simulink model "ADC_forumkerhuel_OC_HW_Fs30k_PIC32"  (Simulink 7.2)
settings: Solver=FixedStepDiscrete  StartTime=0.0  StopTime=inf  FixedStep=1/30000  RelTol=1e-3
undefined symbols (not defined in the file or in its folder): ANmax, OCmax
libraries: dsPICdrivers x4
settings Model: Creator=Lubin  LastModifiedBy=Casparus  BufferReuse=off
settings OptimizationCC: BlockReduction=off  OptimizeBlockIOStorage=off  BufferReuse=off  ExpressionFolding=off  LocalBlockOutputs=off  InitFltsAndDblsToZero=on  OptimizeModelRefInitCode=on  LifeSpan=1
settings DebuggingCC: SaveWithParameterizedLinksMsg=none  SignalResolutionControl=TryResolveAllWithWarning  InheritedTsInSrcMsg=none  IntegerOverflowMsg=none  ParameterOverflowMsg=none
settings HardwareCC: TargetHWDeviceType=32-bit Generic
settings RTWCC: SystemTargetFile=pic32.tlc  TemplateMakefile=pic32_gcc.tmf  PostCodeGenCommand=dsPIC_Compile()  Description=Embedded Target for Microchip dsPIC (real-time)  ProcessScript=pic32_make_rtw_hook
settings CodeAppCC: IgnoreCustomStorageClasses=off
settings STFCustomTargetCC: ModelReferenceCompliant=off  IncludeMdlTerminateFcn=off  CombineOutputUpdateFcns=on  SuppressErrorStatus=on  ERTCustomFileBanners=on  SupportContinuousTime=off  SupportNonInlinedSFcns=off  SystemTargetFile=pic32.tlc
settings ERTTargetCC: MultiwordLength=2048  ModelReferenceCompliant=off  CompOptLevelCompliant=off  IncludeMdlTerminateFcn=off  SuppressErrorStatus=on  ERTFirstTimeCompliant=off  ModelStepFunctionPrototypeControlCompliant=off  CPPClassGenCompliant=off  InlinedParameterPlacement=NonHierarchical  ERTSrcFileBannerTemplate=dsPIC_code_template.cgt  ERTHdrFileBannerTemplate=dsPIC_code_template.cgt  ERTDataSrcFileTemplate=dsPIC_code_template.cgt  ERTDataHdrFileTemplate=dsPIC_code_template.cgt  ERTCustomFileTemplate=dsPIC_main.tlc
settings CustomProperty: DataType=string  Value=C:\PROGRA~1\MATLAB\R2008b\bin\win32\gmake

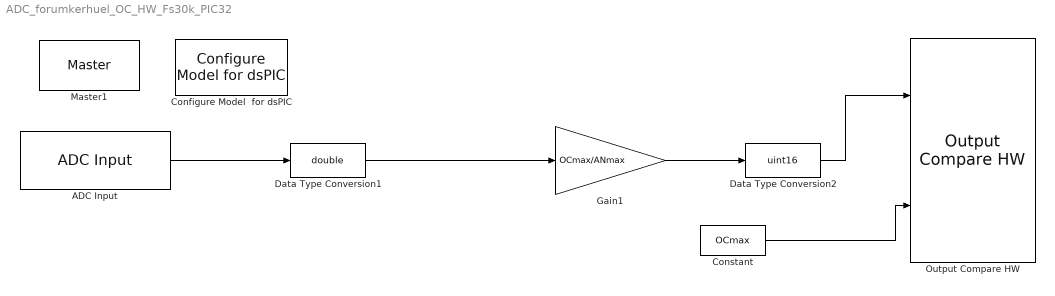
== system ADC_forumkerhuel_OC_HW_Fs30k_PIC32 ==
  ADC Input : dsPICdrivers/Peripheral I//O/ADC Input  Tag=dsPIC_ADC  Priority=5  ADC_TYPE=10 bits  ADC_MODE=Continuous sampling & get last channel value  NbrSampleStep=1  VoltRefpopup="AVdd  -  AVss"  OutFormatBitspopup=0000 00dd dddd dddd : Integer  InterruptPriority=7  ANCHANNELS=[0]  MaxName=ANmax = 1023  Rin=1e2  ADCS=12  SAMC=1  Temperature=25  DMAChannel=0  SampleTime=1/30000  Status="OK  |  Tsmp=1.625e-007 |  T/Channel=2.113e-006 |  Tall=2.113e-006"  SSRC=Timer3 (OC_HW PWM)
  Configure Model  for dsPIC : dsPICdrivers/Simulink Configuration/Configure Model  for dsPIC
  Constant : Constant  Value=OCmax  OutDataTypeMode=uint16  OutDataType=sfix(16)  OutScaling=2^0  OutDataTypeStr=uint16
  Data Type Conversion1 : DataTypeConversion  OutDataTypeMode=double  OutDataType=sfix(16)  OutScaling=2^0  OutDataTypeStr=double
  Data Type Conversion2 : DataTypeConversion  OutDataTypeMode=uint16  OutDataType=sfix(16)  OutScaling=2^0  OutDataTypeStr=uint16
  Gain1 : Gain  Gain=OCmax/ANmax  ParameterDataTypeMode=double  ParameterDataType=sfix(16)  ParameterScaling=2^0  ParamDataTypeStr=double  OutDataType=sfix(16)  OutScaling=2^0
  Master1 : dsPICdrivers/Master  Tag=dsPIC_MASTER  Priority=1  TimeStepType=Free Run  picType=32MX460F512L  fcy=40000000  Quartz_33f=10e6  PLLActive_33f=on  fcyDesired_33f=40000000  tmr1="[1  1332  0.025]"  tmr1Info="Time Step : 3.3325e-005  ;   Error : 0.025%  PR1=1332"  tmr2345="[0  1  0  0]"  tmr2345cfg=[-1 -1 -1 -1]  IOautoConf=on  typePort="[ 0   0   0   0   0   0   0   0   0   0   0   0   0   0   0   0   8   0   0   0   0   0   0   0   0   0   0   0   0   0   0   0   0   0   0   0   0   0   0   0   0   0   0   0   0   0   0   0  24   0   0   0   0   0   0   0   0   0   0   0   0   0   0   0   0   0   0   0   0   0   0   0   0   0   0   0   0   0   0   0   0   0   0   0   0   0   0   0   0   0   0   0   0   0   0   0   0   0   0   0   0   0   0   0   0   0   0   0   0   0   0   0 ]"  TRIS="[ 65535  65535  65535  65534  65535  65535  65535 ]"  ADPCFG=0  MasterBusyPort=None  MasterOverloadPort=None  FOSC=Quartz (XT - HS)  ClockSwitchMonitor=Both disabled  TempProtection_33f=TEMP_ON  FPBOR=<empty>  PWRT=disable  MCLR=<empty>  PowerSave=off  OverrideFcy=off  NewFcy=20e6  PR2345="[65535   1332  65535  65535]"
  Output Compare HW : dsPICdrivers/Peripheral I//O/Output Compare HW  Tag=dsPIC_OC_HW_out  Priority=5  OC_Mode=PWM duty cycle (robust)  Timer=3  CHANNEL=[1]  Channel_UP_Down_Periode=[5]  PeriodeInput=on  MaxChannel=3.3333e-005  MaxName=' OCmax '  Precision=[10.3805]  Status=OK  SafeMarge=[0]  PortLetter=[68]  PortNumber=[0]  MaxValues=[1332]  NPORTS=1
  wires:
  ADC Input/1 -> Data Type Conversion1/1
  Data Type Conversion2/1 -> Output Compare HW/1
  Constant/1 -> Output Compare HW/2
  Gain1/1 -> Data Type Conversion2/1
  Data Type Conversion1/1 -> Gain1/1
